simulink model "AVRsim"  (R2018a)
settings: Solver=ode4  StartTime=starting_time  StopTime=simulation_time  FixedStep=sampling_time  RelTol=1e-3
values from neighbouring files (symbols this model uses):
  Ts = Q.SettlingTime    [PIDAVR.m]
undefined symbols (not defined in the file or in its folder): Kd, Ki, Kp, Ta, Te, Tg
libraries: simulink x22, fod x1
settings Model: Creator=MokRH GameRig  LastModifiedBy=MokRH GameRig

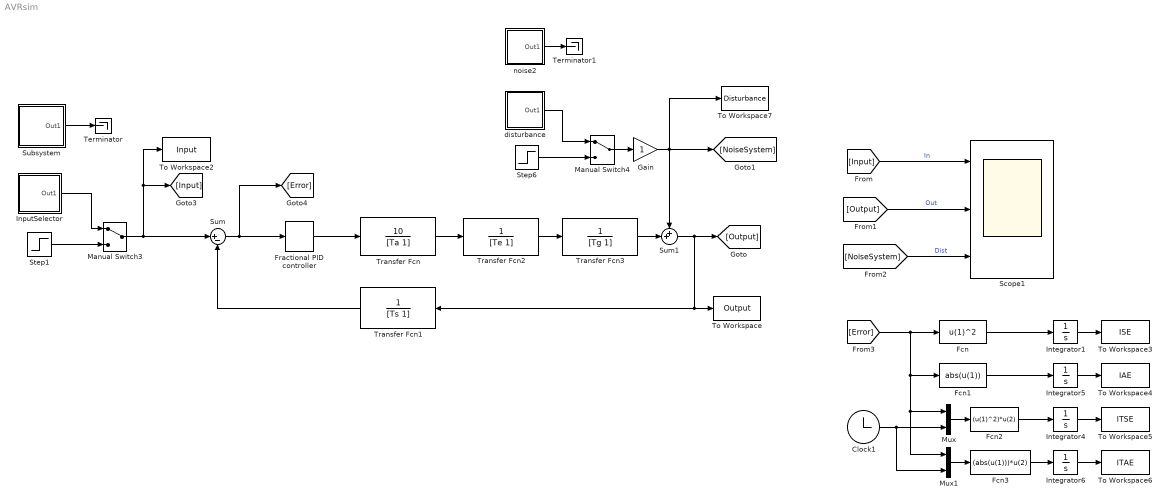
== system AVRsim ==
  Clock1 : Clock
  Fcn : Fcn  Expr=u(1)^2
  Fcn1 : Fcn  Expr=abs(u(1))
  Fcn2 : Fcn  Expr=(u(1)^2)*u(2)
  Fcn3 : Fcn  Expr=(abs(u(1)))*u(2)
  Fractional PID controller : fod/Fractional PID controller  Kp=Kp  Ki=Ki  lambda=lambda  Kd=Kd  mic=mu  freqRange=[1e-4, 1e4]  N=5
      settings: SourceProductName=FOMCON Toolbox
  Gain : Gain
  InputSelector : Subsystem
  Integrator{1,4..6} (4 alike) : Integrator
  Manual Switch3 : ManualSwitch
  Manual Switch4 : ManualSwitch
  Mux : Mux  Inputs=2
  Mux1 : Mux  Inputs=2
  Scope1 : Scope  NumInputPorts=3
  Step1 : Step  Time=0  SampleTime=0.0001
  Step6 : Step  Time=0  After=0  SampleTime=0.0001
  Subsystem : Subsystem
  Sum : Sum  Inputs=|+-
  Sum1 : Sum  Inputs=++|
  Terminator : Terminator
  Terminator1 : Terminator
  To Workspace : ToWorkspace  VariableName=Output  SampleTime=-1
  To Workspace2 : ToWorkspace  VariableName=Input  SampleTime=-1
  To Workspace3 : ToWorkspace  VariableName=ISE  SampleTime=-1
  To Workspace4 : ToWorkspace  VariableName=IAE  SampleTime=-1
  To Workspace5 : ToWorkspace  VariableName=ITSE  SampleTime=-1
  To Workspace6 : ToWorkspace  VariableName=ITAE  SampleTime=-1
  To Workspace7 : ToWorkspace  VariableName=Disturbance  SampleTime=-1
  Transfer Fcn : TransferFcn  Numerator=[10]  Denominator=[Ta 1]
  Transfer Fcn1 : TransferFcn  Denominator=[Ts 1]
  Transfer Fcn2 : TransferFcn  Denominator=[Te 1]
  Transfer Fcn3 : TransferFcn  Denominator=[Tg 1]
  disturbance : Subsystem
  noise2 : Subsystem
  wires:
  Transfer Fcn/1 -> Transfer Fcn2/1
  Transfer Fcn2/1 -> Transfer Fcn3/1
  Transfer Fcn3/1 -> Sum1/2
  Sum1/1 -> [Output], To Workspace/1, Transfer Fcn1/1
  Manual Switch4/1 -> Gain/1
  Mux1/1 -> Fcn3/1
  Integrator6/1 -> To Workspace6/1
  Integrator5/1 -> To Workspace4/1
  Fcn2/1 -> Integrator4/1
  Sum/1 -> Fractional PID controller/1, [Error]
  Integrator1/1 -> To Workspace3/1
  Fcn3/1 -> Integrator6/1
  Fcn1/1 -> Integrator5/1
  Integrator4/1 -> To Workspace5/1
  Fcn/1 -> Integrator1/1
  Mux/1 -> Fcn2/1
  Step6/1 -> Manual Switch4/2
  disturbance/1(Out1) -> Manual Switch4/1
  InputSelector/1(Out1) -> Manual Switch3/1
  Step1/1 -> Manual Switch3/2
  Manual Switch3/1 -> Sum/1, To Workspace2/1, [Input]
  Transfer Fcn1/1 -> Sum/2
  [Output] -> Scope1/2  "Out"
  [Input] -> Scope1/1  "In"
  [NoiseSystem] -> Scope1/3  "Dist"
  Gain/1 -> To Workspace7/1, [NoiseSystem], Sum1/1
  Subsystem/1(Out1) -> Terminator/1
  noise2/1(Out1) -> Terminator1/1
  Fractional PID controller/1 -> Transfer Fcn/1
  [Error] -> Mux1/1, Mux/1, Fcn1/1, Fcn/1
  Clock1/1 -> Mux1/2, Mux/2

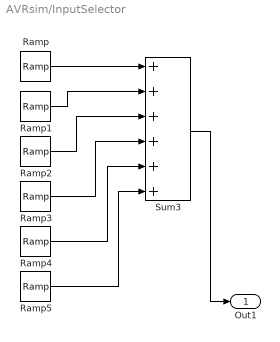
== system AVRsim/InputSelector ==
  Ramp : simulink/Sources/Ramp  slope=1  start=0  InitialOutput=0
  Ramp1 : simulink/Sources/Ramp  slope=-1  start=1  InitialOutput=0
  Ramp2 : simulink/Sources/Ramp  slope=-1  start=2  InitialOutput=0
  Ramp3 : simulink/Sources/Ramp  slope=1  start=4  InitialOutput=0
  Ramp4 : simulink/Sources/Ramp  slope=1  start=5  InitialOutput=0
  Ramp5 : simulink/Sources/Ramp  slope=-1  start=6  InitialOutput=0
  Sum3 : Sum  Inputs=++++++
  Out1 : Outport
  wires:
  Ramp/1 -> Sum3/1
  Ramp4/1 -> Sum3/5
  Ramp1/1 -> Sum3/2
  Ramp3/1 -> Sum3/4
  Ramp5/1 -> Sum3/6
  Ramp2/1 -> Sum3/3
  Sum3/1 -> Out1/1

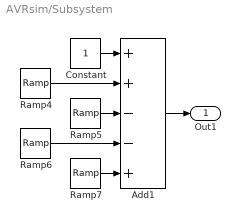
== system AVRsim/Subsystem ==
  Add1 : Sum  Inputs=++--+
  Constant : Constant
  Ramp4 : simulink/Sources/Ramp  slope=2  start=3  InitialOutput=0
  Ramp5 : simulink/Sources/Ramp  slope=2  start=3.5  InitialOutput=0
  Ramp6 : simulink/Sources/Ramp  slope=1  start=6  InitialOutput=0
  Ramp7 : simulink/Sources/Ramp  slope=1  start=7  InitialOutput=0
  Out1 : Outport
  wires:
  Add1/1 -> Out1/1
  Ramp4/1 -> Add1/2
  Ramp7/1 -> Add1/5
  Constant/1 -> Add1/1
  Ramp5/1 -> Add1/3
  Ramp6/1 -> Add1/4

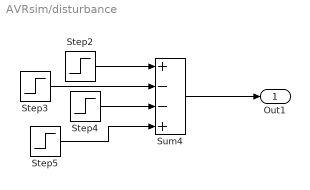
== system AVRsim/disturbance ==
  Step2 : Step  Time=3  SampleTime=0.0001
  Step3 : Step  Time=3.05  SampleTime=0.0001
  Step4 : Step  Time=5.5  SampleTime=0.0001
  Step5 : Step  Time=5.55  SampleTime=0.0001
  Sum4 : Sum  Inputs=+--+
  Out1 : Outport
  wires:
  Step5/1 -> Sum4/4
  Step3/1 -> Sum4/2
  Step4/1 -> Sum4/3
  Step2/1 -> Sum4/1
  Sum4/1 -> Out1/1

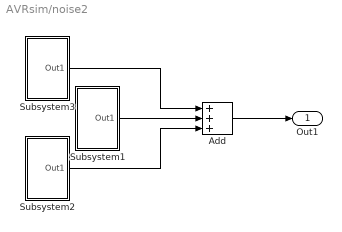
== system AVRsim/noise2 ==
  Add : Sum  Inputs=+++
  Subsystem1 : Subsystem
  Subsystem2 : Subsystem
  Subsystem3 : Subsystem
  Out1 : Outport
  wires:
  Subsystem1/1(Out1) -> Add/2
  Add/1 -> Out1/1
  Subsystem3/1(Out1) -> Add/1
  Subsystem2/1(Out1) -> Add/3

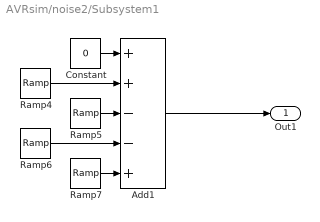
== system AVRsim/noise2/Subsystem1 ==
  Add1 : Sum  Inputs=++--+
  Constant : Constant  Value=0
  Ramp4 : simulink/Sources/Ramp  slope=10  start=4.5  InitialOutput=0
  Ramp5 : simulink/Sources/Ramp  slope=10  start=4.6  InitialOutput=0
  Ramp6 : simulink/Sources/Ramp  slope=5  start=5.3  InitialOutput=0
  Ramp7 : simulink/Sources/Ramp  slope=5  start=5.5  InitialOutput=0
  Out1 : Outport
  wires:
  Ramp5/1 -> Add1/3
  Ramp4/1 -> Add1/2
  Ramp6/1 -> Add1/4
  Constant/1 -> Add1/1
  Ramp7/1 -> Add1/5
  Add1/1 -> Out1/1

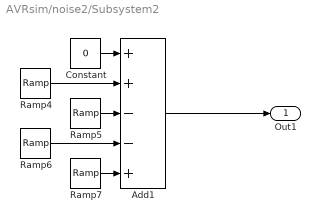
== system AVRsim/noise2/Subsystem2 ==
  Add1 : Sum  Inputs=++--+
  Constant : Constant  Value=0
  Ramp4 : simulink/Sources/Ramp  slope=10  start=6.2  InitialOutput=0
  Ramp5 : simulink/Sources/Ramp  slope=10  start=6.3  InitialOutput=0
  Ramp6 : simulink/Sources/Ramp  slope=5  start=6.6  InitialOutput=0
  Ramp7 : simulink/Sources/Ramp  slope=5  start=6.8  InitialOutput=0
  Out1 : Outport
  wires:
  Ramp5/1 -> Add1/3
  Ramp4/1 -> Add1/2
  Ramp6/1 -> Add1/4
  Constant/1 -> Add1/1
  Ramp7/1 -> Add1/5
  Add1/1 -> Out1/1

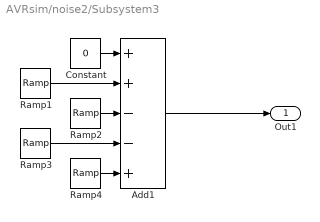
== system AVRsim/noise2/Subsystem3 ==
  Add1 : Sum  Inputs=++--+
  Constant : Constant  Value=0
  Ramp1 : simulink/Sources/Ramp  slope=10  start=3.2  InitialOutput=0
  Ramp2 : simulink/Sources/Ramp  slope=10  start=3.3  InitialOutput=0
  Ramp3 : simulink/Sources/Ramp  slope=5  start=3.6  InitialOutput=0
  Ramp4 : simulink/Sources/Ramp  slope=5  start=3.8  InitialOutput=0
  Out1 : Outport
  wires:
  Ramp2/1 -> Add1/3
  Ramp1/1 -> Add1/2
  Ramp3/1 -> Add1/4
  Constant/1 -> Add1/1
  Ramp4/1 -> Add1/5
  Add1/1 -> Out1/1
